simulink model "hw4_3"  (R2025a)
settings: Solver=VariableStepAuto  StartTime=0.0  StopTime=30  RelTol=1e-3
settings Model: Creator=BCC  LastModifiedBy=BCC

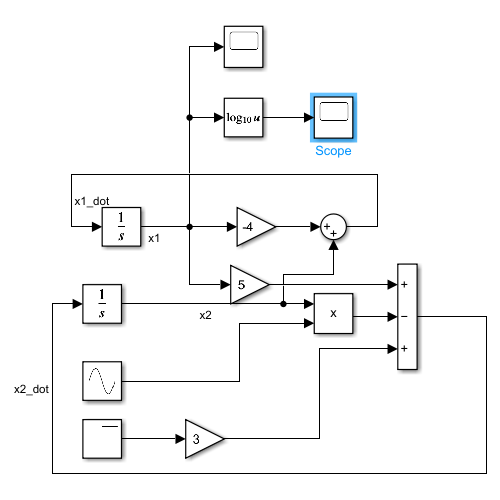
[thumbnail: Simulink's stored preview of the top-level diagram]
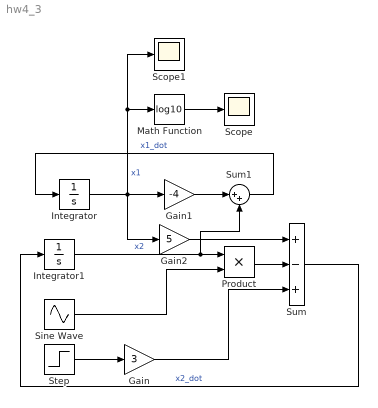
== system hw4_3 ==
  Gain : Gain  Gain=3
  Gain1 : Gain  Gain=-4
  Gain2 : Gain  Gain=5
  Integrator : Integrator
  Integrator1 : Integrator
  Math Function : Math  Operator=log10
  Product : Product
  Scope : Scope
      settings: ActiveDisplayYMinimum=-5.0169595201451767  ActiveDisplayYMaximum=21.333869261833783
  Scope1 : Scope
      settings: ActiveDisplayYMinimum=-9.0862406736625114E+17  ActiveDisplayYMaximum=8.1776166062962627E+18
  Sine Wave : Sin  Amplitude=6  SampleTime=0
  Step : Step  SampleTime=0
  Sum : Sum  Inputs=+-+
  Sum1 : Sum  Inputs=|++
  wires:
  Sum1/1 -> Integrator/1  "x1_dot"
  Integrator/1 -> Math Function/1, Scope1/1, Gain1/1, Gain2/1  "x1"
  Sum/1 -> Integrator1/1  "x2_dot"
  Integrator1/1 -> Sum1/2, Product/1  "x2"
  Sine Wave/1 -> Product/2
  Product/1 -> Sum/2
  Step/1 -> Gain/1
  Gain/1 -> Sum/3
  Gain1/1 -> Sum1/1
  Gain2/1 -> Sum/1
  Math Function/1 -> Scope/1
